simulink model "danxiangbanbozhengliu_R"  (R2025a)
settings: Solver=ode23tb  StartTime=0.0  StopTime=1  MaxStep=1e-5  RelTol=1e-5
libraries: spsACVoltageSourceLib x1, spsDetailedThyristorLib x1, spsMeanLib x1, spsMultimeterLib x1, spsSeriesRLCBranchLib x1, sps_lib x1
settings Model: Creator=小鱼  LastModifiedBy=小鱼

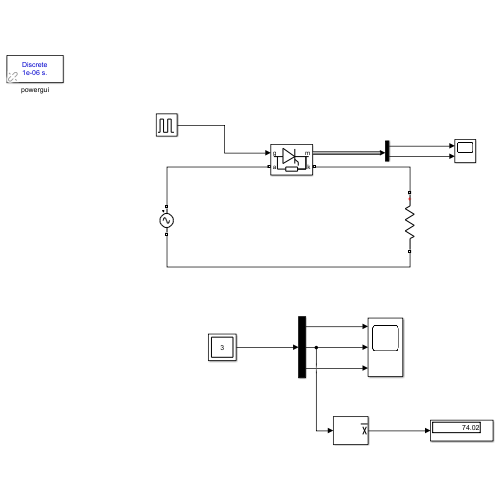
[thumbnail: Simulink's stored preview of the top-level diagram]
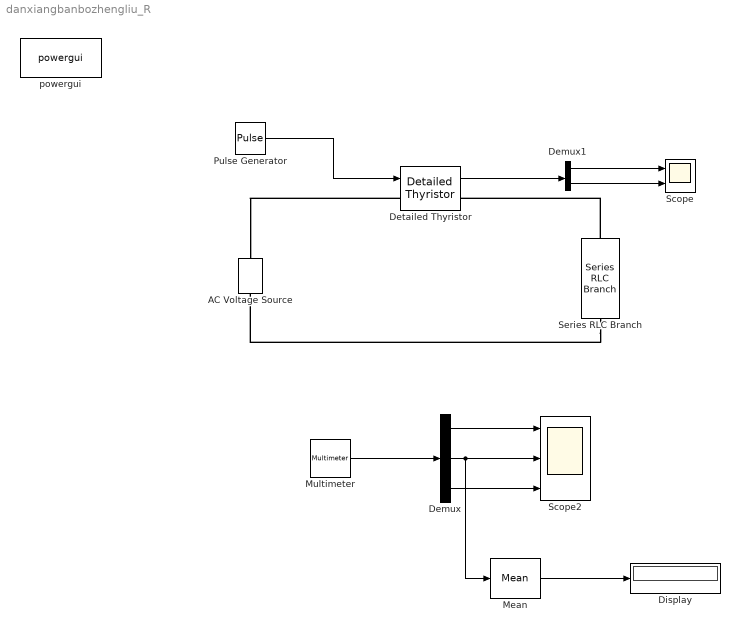
== system danxiangbanbozhengliu_R ==
  AC Voltage Source : spsACVoltageSourceLib/AC Voltage Source  Amplitude=220*sqrt(2)  Phase=0  Frequency=50  SampleTime=0  Measurements=Voltage  BusType=swing  Pref=10e3  Qref=0  Qmin=-inf  Qmax=+inf
  Demux : Demux  Outputs=3
  Demux1 : Demux  Outputs=2
  Detailed Thyristor : spsDetailedThyristorLib/Detailed Thyristor  Ron=0.001  Lon=1e-3  Vf=0.8  IL=0.1  Tq=100e-6  IC=0  Rs=500  Cs=250e-9  Measurements=on
      settings: LibrarySourceBlock=sps_lib/Power Electronics/Detailed Thyristor
  Display : Display
  Mean : spsMeanLib/Mean  Freq=50  Vinit=0  Ts=0
  Multimeter : spsMultimeterLib/Multimeter  L=3  sel=[2 1 3]  yselected={}  Gain=[1 1 1]  OutputType=Complex  PlotAtSimulationStop=off  PhasorSimulation=off
  Pulse Generator : DiscretePulseGenerator  PulseType=Time based  Period=0.02  PulseWidth=5  PhaseDelay=60/360*0.02
  Scope : Scope  NumInputPorts=2
      settings: ActiveDisplayYMinimum=-8.6481217575638674  ActiveDisplayYMaximum=35.878374761920938
  Scope2 : Scope  NumInputPorts=3
      settings: ActiveDisplayYMinimum=-296.76301371803038  ActiveDisplayYMaximum=536.61853617442341  DataLoggingVariableName=ScopeData2
  Series RLC Branch : spsSeriesRLCBranchLib/Series RLC Branch  LConnTagsString=__new0  RConnTagsString=__new0  BranchType=R  Resistance=10  Inductance=1e-3  SetiL0=off  InitialCurrent=0  Capacitance=1e-6  Setx0=off  InitialVoltage=0  Measurements=Branch voltage and current
  powergui : sps_lib/powergui  Priority=1  SimulationMode=Discrete  SampleTime=1e-6  frequency=60  Iterations=50  frequencyindice=50  Pbase=100e6  ErrMax=1e-4  UnitsV=kV  UnitsW=MW  buscounter=0  FunctionMessages=off  echomessages=off  EnableUseOfTLC=off  CurrentSourceSwitches=off  DisableSnubberDevices=off  DisableRonSwitches=off  DisableVfSwitches=off  DisplayEquations=off  AutomaticDiscreteSolvers=off  SolverType=Tustin/Backward Euler (TBE)  Interpol=off  ExternalGateDelay=off  methode=off  Ts=100  x0status=blocks  SPID=on  SwTol=0  HookPort=off  NonlinearTolerance=1e-4  nMaxIteration=100  ContinueOnMaxIteration=off  RestoreLinks=warning  ResistiveCurrentMeasurement=off  Frange=[0:2:500]  Ylog=off  Xlog=on  ShowGrid=off  save=off  variable=ZData  structure=0  ZoomFFT=off  StartTime=0.0  cycles=1  DisplayStyle=1  fundamental=60  FreqAxis=off  MaxFrequency=1000  frequencyindicesteady=1  RmsSteady=1  display=off
  wires:
  Pulse Generator/1 -> Detailed Thyristor/1
  Demux/1 -> Scope2/1
  Demux/3 -> Scope2/3
  Multimeter/1 -> Demux/1
  Demux/2 -> Mean/1, Scope2/2
  Detailed Thyristor/1 -> Demux1/1
  Demux1/1 -> Scope/1
  Demux1/2 -> Scope/2
  Mean/1 -> Display/1
  connections:
  Detailed Thyristor/LConn1 -- AC Voltage Source/RConn1
  Series RLC Branch/LConn1 -- Detailed Thyristor/RConn1
  Series RLC Branch/RConn1 -- AC Voltage Source/LConn1
